simulink model "sistema_fdm_fm"  (R2026a)
settings: Solver=FixedStepDiscrete  StopTime=fuente.T_stop
values from neighbouring files (symbols this model uses):
  P = params_sistema(10e6, o)    [analisis_awgn.m]    (also in graficas_sistema.m = params_sistema(fc_nom, struct('T_real', T_real)); main.m = params_sistema(10e6, struct('imprimir', false)); preparar_entrega.m = params_sistema(10e6, struct('imprimir', false)); probar_audio_real.m = params_sistema(fc_nom, struct('T_real', T_real, 'snr_c_dB', )
undefined symbols (not defined in the file or in its folder): DiscIntNeverNeededParam
Description:
  | Sistema FDM + FM + receptor superheterodino
settings Model: SimulationMode=accelerator  Creator=jordy  LastModifiedBy=jordy

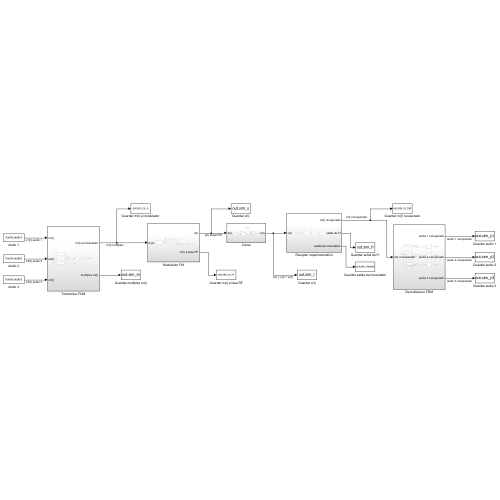
[thumbnail: Simulink's stored preview of the top-level diagram]
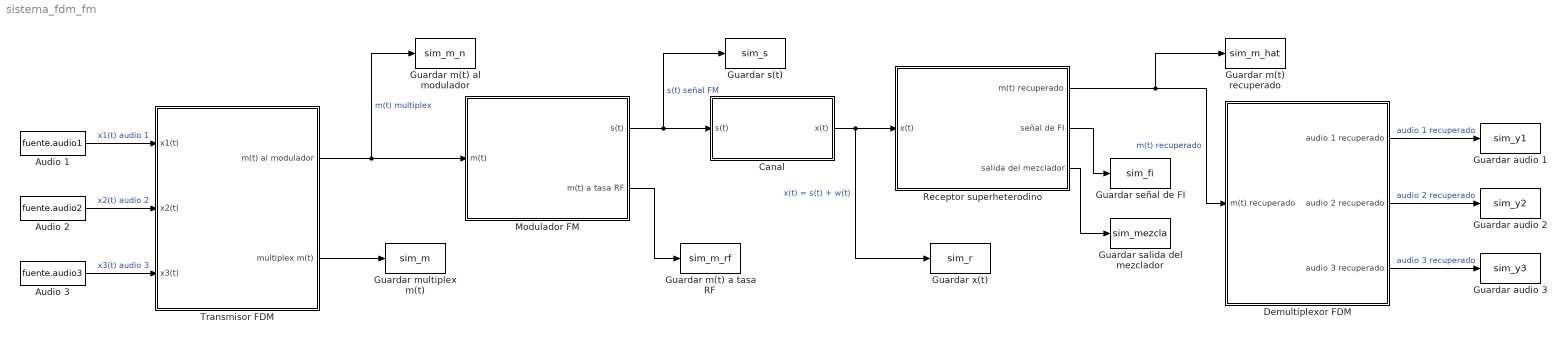
== system sistema_fdm_fm ==
  Audio 1 : FromWorkspace  VariableName=fuente.audio1  SampleTime=1/P.fs_a  Interpolate=off  OutputAfterFinalValue=Setting to zero
  Audio 2 : FromWorkspace  VariableName=fuente.audio2  SampleTime=1/P.fs_a  Interpolate=off  OutputAfterFinalValue=Setting to zero
  Audio 3 : FromWorkspace  VariableName=fuente.audio3  SampleTime=1/P.fs_a  Interpolate=off  OutputAfterFinalValue=Setting to zero
  Canal : Subsystem  Description=r = s + n, n gaussiano de varianza P.sigma_ruido^2 (0 = canal ideal)
  Demultiplexor FDM : Subsystem  Description=Por canal: BPF -> x 2cos(2 pi f_k (t - tau_k)) -> LPF 15 kHz -> decimación a fs_a
  Guardar audio 1 : ToWorkspace  VariableName=sim_y1  SampleTime=-1
  Guardar audio 2 : ToWorkspace  VariableName=sim_y2  SampleTime=-1
  Guardar audio 3 : ToWorkspace  VariableName=sim_y3  SampleTime=-1
  Guardar m(t) a tasa RF : ToWorkspace  VariableName=sim_m_rf  SampleTime=-1
      settings: MaxDataPoints=P.log_rf_max
  Guardar m(t) al modulador : ToWorkspace  VariableName=sim_m_n  SampleTime=-1
  Guardar m(t) recuperado : ToWorkspace  VariableName=sim_m_hat  SampleTime=-1
  Guardar multiplex m(t) : ToWorkspace  VariableName=sim_m  SampleTime=-1
  Guardar s(t) : ToWorkspace  VariableName=sim_s  SampleTime=-1
      settings: MaxDataPoints=P.log_rf_max
  Guardar salida del mezclador : ToWorkspace  VariableName=sim_mezcla  SampleTime=-1
      settings: MaxDataPoints=P.log_rf_max
  Guardar señal de FI : ToWorkspace  VariableName=sim_fi  SampleTime=-1
  Guardar x(t) : ToWorkspace  VariableName=sim_r  SampleTime=-1
      settings: MaxDataPoints=P.log_rf_max
  Modulador FM : Subsystem  Description=Interpolación x100 en dos etapas x10 (fs_m -> fs_fi -> fs_rf) y FM: s = Ac cos(2 pi fc t + 2 pi kf * suma(m_n)/fs_rf)
  Receptor superheterodino : Subsystem  Description=Sección RF (preselector en f_c) -> mezclador con LO = f_c - f_FI -> pasabajos + decimación -> pasabanda FI 1.7 MHz -> demodulador FM en cuadratura -> filtro posdetección -> deénfasis (opcional)
  Transmisor FDM : Subsystem  Description=FDM DSB-SC: LPF 15 kHz, interpolación x10 por inserción de ceros, subportadoras 20/60/100 kHz nom, m_n = m/3, prénfasis (opcional)
  wires:
  Audio 1/1 -> Transmisor FDM/1(x1(t))  "x1(t) audio 1"
  Audio 2/1 -> Transmisor FDM/2(x2(t))  "x2(t) audio 2"
  Audio 3/1 -> Transmisor FDM/3(x3(t))  "x3(t) audio 3"
  Transmisor FDM/2(multiplex m(t)) -> Guardar multiplex m(t)/1
  Transmisor FDM/1(m(t) al modulador) -> Modulador FM/1(m(t)), Guardar m(t) al modulador/1  "m(t) multiplex"
  Modulador FM/2(m(t) a tasa RF) -> Guardar m(t) a tasa RF/1
  Demultiplexor FDM/3(audio 3 recuperado) -> Guardar audio 3/1  "audio 3 recuperado"
  Modulador FM/1(s(t)) -> Canal/1(s(t)), Guardar s(t)/1  "s(t) señal FM"
  Canal/1(x(t)) -> Guardar x(t)/1, Receptor superheterodino/1(x(t))  "x(t) = s(t) + w(t)"
  Receptor superheterodino/1(m(t) recuperado) -> Demultiplexor FDM/1(m(t) recuperado), Guardar m(t) recuperado/1  "m(t) recuperado"
  Receptor superheterodino/2(señal de FI) -> Guardar señal de FI/1
  Receptor superheterodino/3(salida del mezclador) -> Guardar salida del mezclador/1
  Demultiplexor FDM/2(audio 2 recuperado) -> Guardar audio 2/1  "audio 2 recuperado"
  Demultiplexor FDM/1(audio 1 recuperado) -> Guardar audio 1/1  "audio 1 recuperado"

== system sistema_fdm_fm/Canal ==
  s(t) : Inport
  Nivel de ruido : Gain  Gain=P.sigma_ruido
  Ruido blanco gaussiano : RandomNumber  Seed=P.semilla_ruido  SampleTime=1/P.fs_rf
  Suma de ruido w(t) : Sum
  x(t) : Outport
  wires:
  Nivel de ruido/1 -> Suma de ruido w(t)/2
  s(t)/1 -> Suma de ruido w(t)/1
  Ruido blanco gaussiano/1 -> Nivel de ruido/1
  Suma de ruido w(t)/1 -> x(t)/1

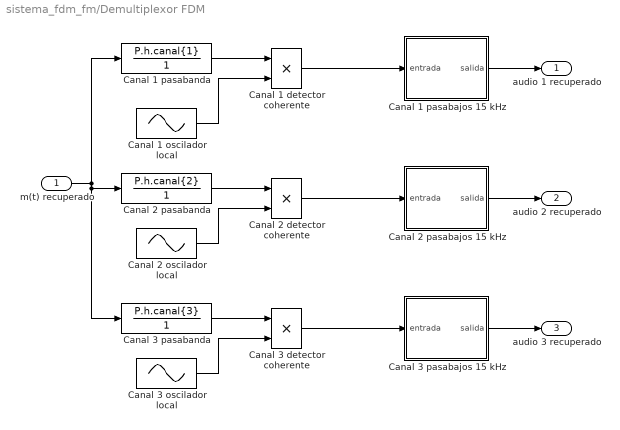
== system sistema_fdm_fm/Demultiplexor FDM ==
  m(t) recuperado : Inport
  Canal 1 detector coherente : Product
  Canal 1 oscilador local : Sin  Amplitude=2  Frequency=2*pi*P.f_sc(1)  Phase=pi/2 + P.fase_rx(1)  SampleTime=1/P.fs_m
  Canal 1 pasabajos 15 kHz : Subsystem
  Canal 1 pasabanda : DiscreteFilter  Numerator=P.h.canal{1}  Denominator=1
  Canal 2 detector coherente : Product
  Canal 2 oscilador local : Sin  Amplitude=2  Frequency=2*pi*P.f_sc(2)  Phase=pi/2 + P.fase_rx(2)  SampleTime=1/P.fs_m
  Canal 2 pasabajos 15 kHz : Subsystem
  Canal 2 pasabanda : DiscreteFilter  Numerator=P.h.canal{2}  Denominator=1
  Canal 3 detector coherente : Product
  Canal 3 oscilador local : Sin  Amplitude=2  Frequency=2*pi*P.f_sc(3)  Phase=pi/2 + P.fase_rx(3)  SampleTime=1/P.fs_m
  Canal 3 pasabajos 15 kHz : Subsystem
  Canal 3 pasabanda : DiscreteFilter  Numerator=P.h.canal{3}  Denominator=1
  audio 1 recuperado : Outport
  audio 2 recuperado : Outport  Port=2
  audio 3 recuperado : Outport  Port=3
  wires:
  m(t) recuperado/1 -> Canal 2 pasabanda/1, Canal 3 pasabanda/1, Canal 1 pasabanda/1
  Canal 1 pasabanda/1 -> Canal 1 detector coherente/1
  Canal 1 oscilador local/1 -> Canal 1 detector coherente/2
  Canal 2 pasabanda/1 -> Canal 2 detector coherente/1
  Canal 2 oscilador local/1 -> Canal 2 detector coherente/2
  Canal 3 pasabanda/1 -> Canal 3 detector coherente/1
  Canal 3 oscilador local/1 -> Canal 3 detector coherente/2
  Canal 1 detector coherente/1 -> Canal 1 pasabajos 15 kHz/1(entrada)
  Canal 1 pasabajos 15 kHz/1(salida) -> audio 1 recuperado/1
  Canal 2 detector coherente/1 -> Canal 2 pasabajos 15 kHz/1(entrada)
  Canal 2 pasabajos 15 kHz/1(salida) -> audio 2 recuperado/1
  Canal 3 detector coherente/1 -> Canal 3 pasabajos 15 kHz/1(entrada)
  Canal 3 pasabajos 15 kHz/1(salida) -> audio 3 recuperado/1

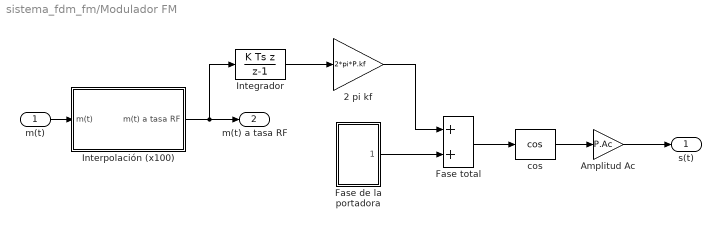
== system sistema_fdm_fm/Modulador FM ==
  m(t) : Inport
  2 pi kf : Gain  Gain=2*pi*P.kf
  Amplitud Ac : Gain  Gain=P.Ac
  Fase de la portadora : Subsystem
  Fase total : Sum
  Integrador : DiscreteIntegrator  IntegratorMethod=Integration: Backward Euler  gainval=1  SampleTime=-1  ICPrevOutput=DiscIntNeverNeededParam  ICPrevScaledInput=DiscIntNeverNeededParam
  Interpolación (x100) : Subsystem
  cos : Trigonometry  Operator=cos
  s(t) : Outport
  m(t) a tasa RF : Outport  Port=2
  wires:
  m(t)/1 -> Interpolación (x100)/1(m(t))
  Interpolación (x100)/1(m(t) a tasa RF) -> Integrador/1, m(t) a tasa RF/1
  Fase total/1 -> cos/1
  2 pi kf/1 -> Fase total/1
  Integrador/1 -> 2 pi kf/1
  Fase de la portadora/1(2 pi fc t) -> Fase total/2
  Amplitud Ac/1 -> s(t)/1
  cos/1 -> Amplitud Ac/1

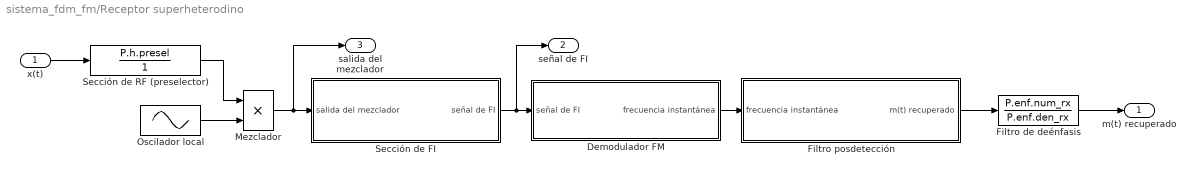
== system sistema_fdm_fm/Receptor superheterodino ==
  x(t) : Inport
  Demodulador FM : Subsystem  Description=Discriminador: limitador (normaliza la amplitud) -> detector de pendiente (derivador) -> detector de envolvente (ley cuadrática).
  Filtro de deénfasis : DiscreteFilter  Description=Deénfasis H(z) = (1/g)/(1 - a z^-1): devuelve el multiplex a su forma original y atenúa el ruido de alta frecuencia  Numerator=P.enf.num_rx  Denominator=P.enf.den_rx
  Filtro posdetección : Subsystem
  Mezclador : Product
  Oscilador local : Sin  Amplitude=2  Frequency=2*pi*P.f_LO  Phase=pi/2  SampleTime=1/P.fs_rf
  Sección de FI : Subsystem
  Sección de RF (preselector) : DiscreteFilter  Numerator=P.h.presel  Denominator=1
  m(t) recuperado : Outport
  señal de FI : Outport  Port=2
  salida del mezclador : Outport  Port=3
  wires:
  Mezclador/1 -> salida del mezclador/1, Sección de FI/1(salida del mezclador)
  Oscilador local/1 -> Mezclador/2
  Sección de RF (preselector)/1 -> Mezclador/1
  x(t)/1 -> Sección de RF (preselector)/1
  Filtro posdetección/1(m(t) recuperado) -> Filtro de deénfasis/1
  Demodulador FM/1(frecuencia instantánea) -> Filtro posdetección/1(frecuencia instantánea)
  Sección de FI/1(señal de FI) -> Demodulador FM/1(señal de FI), señal de FI/1
  Filtro de deénfasis/1 -> m(t) recuperado/1

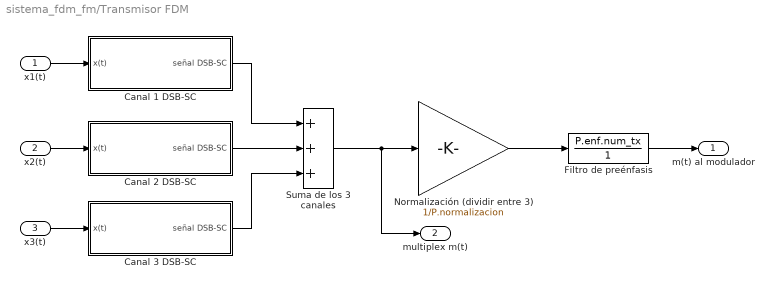
== system sistema_fdm_fm/Transmisor FDM ==
  x1(t) : Inport
  x2(t) : Inport  Port=2
  x3(t) : Inport  Port=3
  Canal 1 DSB-SC : Subsystem  Description=Canal 1: DSB-SC con subportadora P.f_sc(1). Interpolación x P.L1 = Rate Transition (retención) x tren de pulsos -> inserción de ceros; luego FIR con ganancia L1.
  Canal 2 DSB-SC : Subsystem  Description=Canal 2: DSB-SC con subportadora P.f_sc(2). Interpolación x P.L1 = Rate Transition (retención) x tren de pulsos -> inserción de ceros; luego FIR con ganancia L1.
  Canal 3 DSB-SC : Subsystem  Description=Canal 3: DSB-SC con subportadora P.f_sc(3). Interpolación x P.L1 = Rate Transition (retención) x tren de pulsos -> inserción de ceros; luego FIR con ganancia L1.
  Filtro de preénfasis : DiscreteFilter  Description=Prénfasis H(z) = g (1 - a z^-1): realza los canales altos antes del modulador FM  Numerator=P.enf.num_tx  Denominator=1
  Normalización (dividir entre 3) : Gain  Gain=1/P.normalizacion
  Suma de los 3 canales : Sum  Inputs=+++
  m(t) al modulador : Outport
  multiplex m(t) : Outport  Port=2
  wires:
  Canal 1 DSB-SC/1(señal DSB-SC) -> Suma de los 3 canales/1
  x1(t)/1 -> Canal 1 DSB-SC/1(x(t))
  x2(t)/1 -> Canal 2 DSB-SC/1(x(t))
  Canal 2 DSB-SC/1(señal DSB-SC) -> Suma de los 3 canales/2
  x3(t)/1 -> Canal 3 DSB-SC/1(x(t))
  Canal 3 DSB-SC/1(señal DSB-SC) -> Suma de los 3 canales/3
  Suma de los 3 canales/1 -> Normalización (dividir entre 3)/1, multiplex m(t)/1
  Filtro de preénfasis/1 -> m(t) al modulador/1
  Normalización (dividir entre 3)/1 -> Filtro de preénfasis/1

== system sistema_fdm_fm/Demultiplexor FDM/Canal 1 pasabajos 15 kHz ==
  entrada : Inport
  Bajar tasa 10 a 1 : RateTransition  Deterministic=off  OutPortSampleTime=1/P.fs_a
  Pasabajos 15 kHz : DiscreteFilter  Numerator=P.h.post  Denominator=1
  salida : Outport
  wires:
  entrada/1 -> Pasabajos 15 kHz/1
  Pasabajos 15 kHz/1 -> Bajar tasa 10 a 1/1
  Bajar tasa 10 a 1/1 -> salida/1

== system sistema_fdm_fm/Demultiplexor FDM/Canal 2 pasabajos 15 kHz ==
  entrada : Inport
  Bajar tasa 10 a 1 : RateTransition  Deterministic=off  OutPortSampleTime=1/P.fs_a
  Pasabajos 15 kHz : DiscreteFilter  Numerator=P.h.post  Denominator=1
  salida : Outport
  wires:
  entrada/1 -> Pasabajos 15 kHz/1
  Pasabajos 15 kHz/1 -> Bajar tasa 10 a 1/1
  Bajar tasa 10 a 1/1 -> salida/1

== system sistema_fdm_fm/Demultiplexor FDM/Canal 3 pasabajos 15 kHz ==
  entrada : Inport
  Bajar tasa 10 a 1 : RateTransition  Deterministic=off  OutPortSampleTime=1/P.fs_a
  Pasabajos 15 kHz : DiscreteFilter  Numerator=P.h.post  Denominator=1
  salida : Outport
  wires:
  Pasabajos 15 kHz/1 -> Bajar tasa 10 a 1/1
  Bajar tasa 10 a 1/1 -> salida/1
  entrada/1 -> Pasabajos 15 kHz/1

== system sistema_fdm_fm/Modulador FM/Fase de la portadora ==
  2 pi fc : Gain  Gain=2*pi*P.fc
  Reloj t : DigitalClock  SampleTime=1/P.fs_rf
  2 pi fc t : Outport
  wires:
  2 pi fc/1 -> 2 pi fc t/1
  Reloj t/1 -> 2 pi fc/1

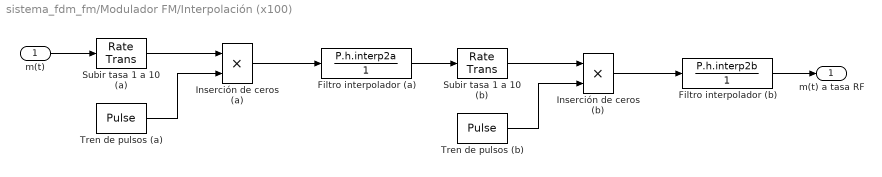
== system sistema_fdm_fm/Modulador FM/Interpolación (x100) ==
  m(t) : Inport
  Filtro interpolador (a) : DiscreteFilter  Numerator=P.h.interp2a  Denominator=1
  Filtro interpolador (b) : DiscreteFilter  Numerator=P.h.interp2b  Denominator=1
  Inserción de ceros (a) : Product
  Inserción de ceros (b) : Product
  Subir tasa 1 a 10 (a) : RateTransition  Deterministic=off  OutPortSampleTime=1/P.fs_fi
  Subir tasa 1 a 10 (b) : RateTransition  Deterministic=off  OutPortSampleTime=1/P.fs_rf
  Tren de pulsos (a) : DiscretePulseGenerator  Period=P.L2a  SampleTime=1/P.fs_fi
  Tren de pulsos (b) : DiscretePulseGenerator  Period=P.L2b  SampleTime=1/P.fs_rf
  m(t) a tasa RF : Outport
  wires:
  m(t)/1 -> Subir tasa 1 a 10 (a)/1
  Inserción de ceros (b)/1 -> Filtro interpolador (b)/1
  Filtro interpolador (a)/1 -> Subir tasa 1 a 10 (b)/1
  Tren de pulsos (b)/1 -> Inserción de ceros (b)/2
  Subir tasa 1 a 10 (b)/1 -> Inserción de ceros (b)/1
  Inserción de ceros (a)/1 -> Filtro interpolador (a)/1
  Tren de pulsos (a)/1 -> Inserción de ceros (a)/2
  Subir tasa 1 a 10 (a)/1 -> Inserción de ceros (a)/1
  Filtro interpolador (b)/1 -> m(t) a tasa RF/1

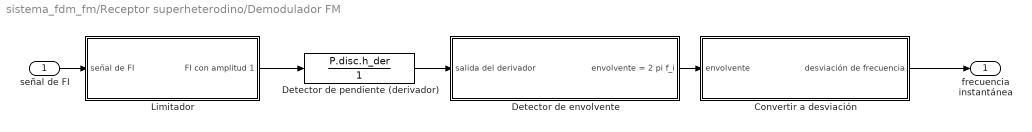
== system sistema_fdm_fm/Receptor superheterodino/Demodulador FM ==
  señal de FI : Inport
  Convertir a desviación : Subsystem
  Detector de envolvente : Subsystem
  Detector de pendiente (derivador) : DiscreteFilter  Numerator=P.disc.h_der  Denominator=1
  Limitador : Subsystem
  frecuencia instantánea : Outport
  wires:
  señal de FI/1 -> Limitador/1(señal de FI)
  Convertir a desviación/1(desviación de frecuencia) -> frecuencia instantánea/1
  Detector de envolvente/1(envolvente = 2 pi f_i) -> Convertir a desviación/1(envolvente)
  Limitador/1(FI con amplitud 1) -> Detector de pendiente (derivador)/1
  Detector de pendiente (derivador)/1 -> Detector de envolvente/1(salida del derivador)

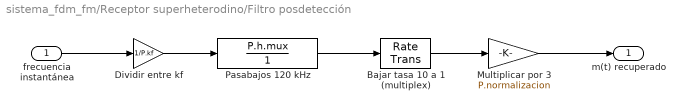
== system sistema_fdm_fm/Receptor superheterodino/Filtro posdetección ==
  frecuencia instantánea : Inport
  Bajar tasa 10 a 1 (multiplex) : RateTransition  Deterministic=off  OutPortSampleTime=1/P.fs_m
  Dividir entre kf : Gain  Gain=1/P.kf
  Multiplicar por 3 : Gain  Gain=P.normalizacion
  Pasabajos 120 kHz : DiscreteFilter  Numerator=P.h.mux  Denominator=1
  m(t) recuperado : Outport
  wires:
  Multiplicar por 3/1 -> m(t) recuperado/1
  Bajar tasa 10 a 1 (multiplex)/1 -> Multiplicar por 3/1
  Pasabajos 120 kHz/1 -> Bajar tasa 10 a 1 (multiplex)/1
  Dividir entre kf/1 -> Pasabajos 120 kHz/1
  frecuencia instantánea/1 -> Dividir entre kf/1

== system sistema_fdm_fm/Receptor superheterodino/Sección de FI ==
  salida del mezclador : Inport
  Bajar tasa 10 a 1 (FI) : RateTransition  Deterministic=off  OutPortSampleTime=1/P.fs_fi
  Filtro antitraslape : DiscreteFilter  Numerator=P.h.fi_lpf  Denominator=1
  Pasabanda de FI : DiscreteFilter  Numerator=P.h.fi  Denominator=1
  señal de FI : Outport
  wires:
  salida del mezclador/1 -> Filtro antitraslape/1
  Bajar tasa 10 a 1 (FI)/1 -> Pasabanda de FI/1
  Filtro antitraslape/1 -> Bajar tasa 10 a 1 (FI)/1
  Pasabanda de FI/1 -> señal de FI/1

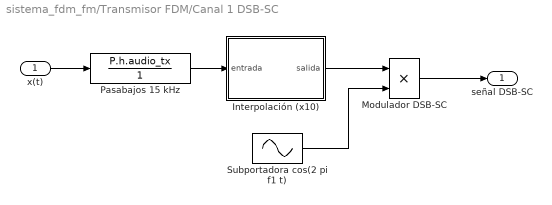
== system sistema_fdm_fm/Transmisor FDM/Canal 1 DSB-SC ==
  x(t) : Inport
  Interpolación (x10) : Subsystem
  Modulador DSB-SC : Product
  Pasabajos 15 kHz : DiscreteFilter  Numerator=P.h.audio_tx  Denominator=1
  Subportadora cos(2 pi f1 t) : Sin  Frequency=2*pi*P.f_sc(1)  Phase=pi/2  SampleTime=1/P.fs_m
  señal DSB-SC : Outport
  wires:
  Modulador DSB-SC/1 -> señal DSB-SC/1
  x(t)/1 -> Pasabajos 15 kHz/1
  Pasabajos 15 kHz/1 -> Interpolación (x10)/1(entrada)
  Interpolación (x10)/1(salida) -> Modulador DSB-SC/1
  Subportadora cos(2 pi f1 t)/1 -> Modulador DSB-SC/2

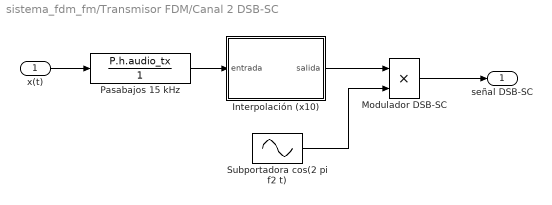
== system sistema_fdm_fm/Transmisor FDM/Canal 2 DSB-SC ==
  x(t) : Inport
  Interpolación (x10) : Subsystem
  Modulador DSB-SC : Product
  Pasabajos 15 kHz : DiscreteFilter  Numerator=P.h.audio_tx  Denominator=1
  Subportadora cos(2 pi f2 t) : Sin  Frequency=2*pi*P.f_sc(2)  Phase=pi/2  SampleTime=1/P.fs_m
  señal DSB-SC : Outport
  wires:
  Pasabajos 15 kHz/1 -> Interpolación (x10)/1(entrada)
  x(t)/1 -> Pasabajos 15 kHz/1
  Interpolación (x10)/1(salida) -> Modulador DSB-SC/1
  Modulador DSB-SC/1 -> señal DSB-SC/1
  Subportadora cos(2 pi f2 t)/1 -> Modulador DSB-SC/2

== system sistema_fdm_fm/Transmisor FDM/Canal 3 DSB-SC ==
  x(t) : Inport
  Interpolación (x10) : Subsystem
  Modulador DSB-SC : Product
  Pasabajos 15 kHz : DiscreteFilter  Numerator=P.h.audio_tx  Denominator=1
  Subportadora cos(2 pi f3 t) : Sin  Frequency=2*pi*P.f_sc(3)  Phase=pi/2  SampleTime=1/P.fs_m
  señal DSB-SC : Outport
  wires:
  x(t)/1 -> Pasabajos 15 kHz/1
  Subportadora cos(2 pi f3 t)/1 -> Modulador DSB-SC/2
  Pasabajos 15 kHz/1 -> Interpolación (x10)/1(entrada)
  Modulador DSB-SC/1 -> señal DSB-SC/1
  Interpolación (x10)/1(salida) -> Modulador DSB-SC/1

== system sistema_fdm_fm/Receptor superheterodino/Demodulador FM/Convertir a desviación ==
  envolvente : Inport
  Dividir entre 2 pi : Gain  Gain=1/(2*pi)
  Frecuencia de FI : Constant  Value=P.f_FI
  Restar la FI : Sum  Inputs=+-
  desviación de frecuencia : Outport
  wires:
  envolvente/1 -> Dividir entre 2 pi/1
  Restar la FI/1 -> desviación de frecuencia/1
  Frecuencia de FI/1 -> Restar la FI/2
  Dividir entre 2 pi/1 -> Restar la FI/1

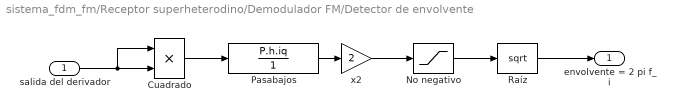
== system sistema_fdm_fm/Receptor superheterodino/Demodulador FM/Detector de envolvente ==
  salida del derivador : Inport
  Cuadrado : Product
  No negativo : Saturate  UpperLimit=inf  LowerLimit=0
  Pasabajos : DiscreteFilter  Numerator=P.h.iq  Denominator=1
  Raíz : Sqrt
  x2 : Gain  Gain=2
  envolvente = 2 pi f_i : Outport
  wires:
  salida del derivador/1 -> Cuadrado/1, Cuadrado/2
  Raíz/1 -> envolvente = 2 pi f_i/1
  No negativo/1 -> Raíz/1
  x2/1 -> No negativo/1
  Pasabajos/1 -> x2/1
  Cuadrado/1 -> Pasabajos/1

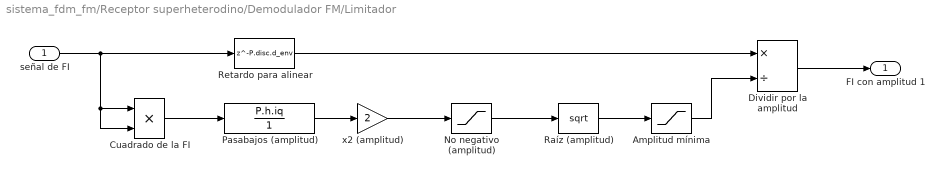
== system sistema_fdm_fm/Receptor superheterodino/Demodulador FM/Limitador ==
  señal de FI : Inport
  Amplitud mínima : Saturate  UpperLimit=inf  LowerLimit=P.disc.amin
  Cuadrado de la FI : Product
  Dividir por la amplitud : Product  Inputs=*/
  No negativo (amplitud) : Saturate  UpperLimit=inf  LowerLimit=0
  Pasabajos (amplitud) : DiscreteFilter  Numerator=P.h.iq  Denominator=1
  Raíz (amplitud) : Sqrt
  Retardo para alinear : Delay  DelayLength=P.disc.d_env  InitialCondition=0
  x2 (amplitud) : Gain  Gain=2
  FI con amplitud 1 : Outport
  wires:
  señal de FI/1 -> Cuadrado de la FI/2, Cuadrado de la FI/1, Retardo para alinear/1
  Amplitud mínima/1 -> Dividir por la amplitud/2
  Raíz (amplitud)/1 -> Amplitud mínima/1
  No negativo (amplitud)/1 -> Raíz (amplitud)/1
  x2 (amplitud)/1 -> No negativo (amplitud)/1
  Pasabajos (amplitud)/1 -> x2 (amplitud)/1
  Cuadrado de la FI/1 -> Pasabajos (amplitud)/1
  Dividir por la amplitud/1 -> FI con amplitud 1/1
  Retardo para alinear/1 -> Dividir por la amplitud/1

== system sistema_fdm_fm/Transmisor FDM/Canal 1 DSB-SC/Interpolación (x10) ==
  entrada : Inport
  Filtro interpolador : DiscreteFilter  Numerator=P.h.interp1  Denominator=1
  Inserción de ceros : Product
  Subir tasa 1 a 10 : RateTransition  Deterministic=off  OutPortSampleTime=1/P.fs_m
  Tren de pulsos : DiscretePulseGenerator  Period=P.L1  SampleTime=1/P.fs_m
  salida : Outport
  wires:
  Subir tasa 1 a 10/1 -> Inserción de ceros/1
  entrada/1 -> Subir tasa 1 a 10/1
  Tren de pulsos/1 -> Inserción de ceros/2
  Filtro interpolador/1 -> salida/1
  Inserción de ceros/1 -> Filtro interpolador/1

== system sistema_fdm_fm/Transmisor FDM/Canal 2 DSB-SC/Interpolación (x10) ==
  entrada : Inport
  Filtro interpolador : DiscreteFilter  Numerator=P.h.interp1  Denominator=1
  Inserción de ceros : Product
  Subir tasa 1 a 10 : RateTransition  Deterministic=off  OutPortSampleTime=1/P.fs_m
  Tren de pulsos : DiscretePulseGenerator  Period=P.L1  SampleTime=1/P.fs_m
  salida : Outport
  wires:
  entrada/1 -> Subir tasa 1 a 10/1
  Tren de pulsos/1 -> Inserción de ceros/2
  Subir tasa 1 a 10/1 -> Inserción de ceros/1
  Filtro interpolador/1 -> salida/1
  Inserción de ceros/1 -> Filtro interpolador/1

== system sistema_fdm_fm/Transmisor FDM/Canal 3 DSB-SC/Interpolación (x10) ==
  entrada : Inport
  Filtro interpolador : DiscreteFilter  Numerator=P.h.interp1  Denominator=1
  Inserción de ceros : Product
  Subir tasa 1 a 10 : RateTransition  Deterministic=off  OutPortSampleTime=1/P.fs_m
  Tren de pulsos : DiscretePulseGenerator  Period=P.L1  SampleTime=1/P.fs_m
  salida : Outport
  wires:
  entrada/1 -> Subir tasa 1 a 10/1
  Filtro interpolador/1 -> salida/1
  Inserción de ceros/1 -> Filtro interpolador/1
  Tren de pulsos/1 -> Inserción de ceros/2
  Subir tasa 1 a 10/1 -> Inserción de ceros/1
